simulink model "DSimulator_abbIRB4v2"  (R2021a)
settings: Solver=ode1  StartTime=0.0  StopTime=30  FixedStep=0.001  RelTol=1e-3  EnableMultiTasking=on
undefined symbols (not defined in the file or in its folder): plotRobot_dynamic
CloseFcn:
  | EraseHandles
Description:
  | Dynamic Simulator robot ABB IRB120 4DOF (Load Parameters from file)
settings Model: NumberOfSteps=5  Creator=E. Dean  LastModifiedBy=little_long
settings SolverCC: AlgebraicLoopSolver=TrustRegion
settings DataIOCC: LimitDataPoints=on  SaveFormat=Array  SignalLoggingSaveFormat=ModelDataLogs  ReturnWorkspaceOutputs=off
settings OptimizationCC: ExpressionDepthLimit=2147483647  LifeSpan=inf
settings DebuggingCC: UnderspecifiedInitializationDetection=Classic  MergeDetectMultiDrivingBlocksExec=none  SolverPrmCheckMsg=warning  FcnCallInpInsideContextMsg=warning  StateNameClashWarn=warning  SFUnexpectedBacktrackingDiag=warning  SFNoUnconditionalDefaultTransitionDiag=warning  SFExecutionAtInitializationDiag=none  SFMachineParentedDataDiag=warning  ArithmeticOperatorsInVariantConditions=warning
settings HardwareCC: ProdBitPerPointer=32  ProdBitPerSizeT=32  ProdBitPerPtrDiffT=32  ProdLargestAtomicFloat=None  ProdIntDivRoundTo=Undefined  ProdEndianess=Unspecified  ProdWordSize=32  ProdHWDeviceType=32-bit Generic
settings ModelReferenceCC: PropagateSignalLabelsOutOfModel=off
settings SFSimCC: SimUseLocalCustomCode=off  CustomCodeUndefinedFunction=UseInterfaceOnly
settings RTWCC: RTWUseLocalCustomCode=off
settings CodeAppCC: StateflowObjectComments=on
settings GRTTargetCC: TargetLangStandard=C89/C90 (ANSI)  CombineOutputUpdateFcns=off  GRTInterface=on
settings ConfigComp: CovMetricSettings=dw  CovSaveCumulativeToWorkspaceVar=on  CovSaveSingleToWorkspaceVar=on

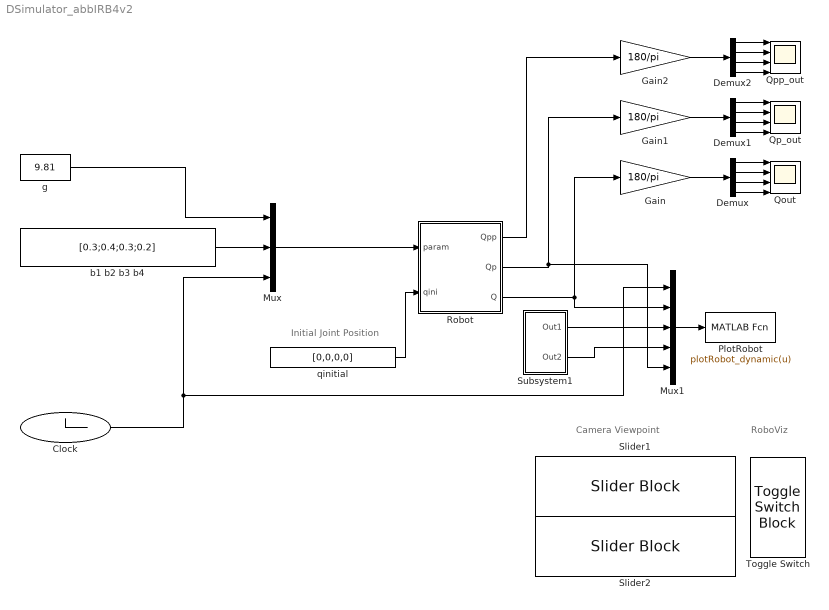
== system DSimulator_abbIRB4v2 ==
  note: Initial Joint Position
  note: Camera Viewpoint
  note: RoboViz
  Clock : Clock
  Demux : Demux
  Demux1 : Demux
  Demux2 : Demux
  Gain : Gain  Gain=180/pi
  Gain1 : Gain  Gain=180/pi
  Gain2 : Gain  Gain=180/pi
  Mux : Mux  Inputs=3
  Mux1 : Mux  Inputs=[1, 4, 2, 1, 4]
  PlotRobot : MATLABFcn  MATLABFcn=plotRobot_dynamic(u)  OutputDimensions=0
  Qout : Scope  NumInputPorts=4
  Qp_out : Scope  NumInputPorts=4
  Qpp_out : Scope  NumInputPorts=4
  Robot : Subsystem
  Slider1 : SliderBlock  ScaleMin=-180  ScaleMax=180  TickInterval=180
  Slider2 : SliderBlock  ScaleMin=-180  ScaleMax=180  TickInterval=180
  Subsystem1 : Subsystem
  Toggle Switch : ToggleSwitchBlock
      settings: Values={{'Off', 'On'}, [0 1]}
  "b1 b2 b3 b4 " : Constant  Value=[0.3;0.4;0.3;0.2]
  g : Constant  Value=9.81
  qinitial : Constant  Value=[0,0,0,0]
  wires:
  Gain/1 -> Demux/1
  Demux/1 -> Qout/1
  Demux/2 -> Qout/2
  Demux/3 -> Qout/3
  Gain1/1 -> Demux1/1
  Demux1/1 -> Qp_out/1
  Demux1/2 -> Qp_out/2
  Demux1/3 -> Qp_out/3
  Demux1/4 -> Qp_out/4
  g/1 -> Mux/1
  Clock/1 -> Mux/3, Mux1/1
  Mux1/1 -> PlotRobot/1
  Demux/4 -> Qout/4
  Demux2/1 -> Qpp_out/1
  Demux2/2 -> Qpp_out/2
  Demux2/3 -> Qpp_out/3
  Gain2/1 -> Demux2/1
  Demux2/4 -> Qpp_out/4
  Robot/3(Q) -> Gain/1, Mux1/2
  Robot/2(Qp) -> Mux1/5, Gain1/1
  Mux/1 -> Robot/1(param)
  qinitial/1 -> Robot/2(qini)
  Robot/1(Qpp) -> Gain2/1
  "b1 b2 b3 b4 "/1 -> Mux/2
  Subsystem1/1(Out1) -> Mux1/3
  Subsystem1/2(Out2) -> Mux1/4

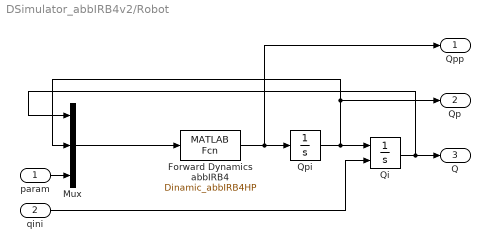
== system DSimulator_abbIRB4v2/Robot ==
  param : Inport
  qini : Inport  Port=2
  Forward Dynamics abbIRB4 : MATLABFcn  MATLABFcn=Dinamic_abbIRB4HP  OutputDimensions=4
  Mux : Mux  Inputs=3
  Qi : Integrator  InitialConditionSource=external  InitialCondition=[0;0;0;0]
  Qpi : Integrator  InitialCondition=[0;0;0;0]
  Qpp : Outport
  Qp : Outport  Port=2
  Q : Outport  Port=3
  wires:
  Qi/1 -> Mux/1, Q/1
  qini/1 -> Qi/2
  Forward Dynamics abbIRB4/1 -> Qpp/1, Qpi/1
  Qpi/1 -> Mux/2, Qp/1, Qi/1
  param/1 -> Mux/3
  Mux/1 -> Forward Dynamics abbIRB4/1

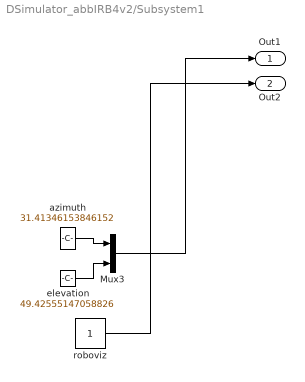
== system DSimulator_abbIRB4v2/Subsystem1 ==
  Mux3 : Mux  Inputs=2
  azimuth : Constant  Value=31.41346153846152
  elevation : Constant  Value=49.42555147058826
  roboviz : Constant
  Out1 : Outport
  Out2 : Outport  Port=2
  wires:
  azimuth/1 -> Mux3/1
  roboviz/1 -> Out2/1
  elevation/1 -> Mux3/2
  Mux3/1 -> Out1/1
